simulink model "ARIES"  (R2024b)
settings: Solver=ode4  StartTime=0.0  StopTime=8*18601.8746  FixedStep=1e-1  RelTol=1e-3
model workspace (MAT data in the model file):
  BVH_bboxMax = Simulink.Parameter
  BVH_bboxMax.Value = [284.93805 4.355131 284.93805 278.0491 284.93805 284.65656 284.93805 139.47609 284.93805 284.93805 268.4671 268.4671 ... (24573 elements, 8191x3)]
  BVH_bboxMax.Complexity = 'real'
  BVH_bboxMax.Dimensions = [8191 3]
  BVH_bboxMax.DataType = 'auto'
  BVH_bboxMin = Simulink.Parameter
  BVH_bboxMin.Value = [-277.88974 -277.88974 -8.175628 -8.175628 -7.5725703 -7.2454505 -7.5725703 -7.5725703 128.49397 129.55234 128.49397 128.49397 ... (24573 elements, 8191x3)]
  BVH_bboxMin.Complexity = 'real'
  BVH_bboxMin.Dimensions = [8191 3]
  BVH_bboxMin.DataType = 'auto'
  BVH_fCount = Simulink.Parameter
  BVH_fCount.Value = [0 0 0 0 0 0 0 0 0 0 0 0 ... (8191 elements, 8191x1)]
  BVH_fCount.Complexity = 'real'
  BVH_fCount.Dimensions = [8191 1]
  BVH_fCount.DataType = 'int32'
  BVH_fStart = Simulink.Parameter
  BVH_fStart.Value = [0 0 0 0 0 0 0 0 0 0 0 0 ... (8191 elements, 8191x1)]
  BVH_fStart.Complexity = 'real'
  BVH_fStart.Dimensions = [8191 1]
  BVH_fStart.DataType = 'int32'
  BVH_faces = Simulink.Parameter
  BVH_faces.Value = [6744 6709 6709 6698 6730 6729 6745 6681 6682 6684 6684 6682 ... (74994 elements, 24998x3)]
  BVH_faces.Complexity = 'real'
  BVH_faces.Dimensions = [24998 3]
  BVH_faces.DataType = 'int32'
  BVH_left = Simulink.Parameter
  BVH_left.Value = [2 4098 4 2052 6 1030 8 520 10 266 12 140 ... (8191 elements, 8191x1)]
  BVH_left.Complexity = 'real'
  BVH_left.Dimensions = [8191 1]
  BVH_left.DataType = 'int32'
  BVH_normals = Simulink.Parameter
  BVH_normals.Value = [1 1 1 1 1 1 0 1 1 1 1 1 ... (74994 elements, 24998x3)]
  BVH_normals.Complexity = 'real'
  BVH_normals.Dimensions = [24998 3]
  BVH_normals.DataType = 'auto'
  BVH_right = Simulink.Parameter
  BVH_right.Value = [3 4099 5 2053 7 1031 9 521 11 267 13 141 ... (8191 elements, 8191x1)]
  BVH_right.Complexity = 'real'
  BVH_right.Dimensions = [8191 1]
  BVH_right.DataType = 'int32'
  BVH_vertexList = Simulink.Parameter
  BVH_vertexList.Value = [-118.90262 -122.20188 -116.06995 -125.190315 -127.74983 -122.412506 -131.21611 -134.88121 -129.40932 -138.59775 -133.93816 -136.61743 ... (37503 elements, 12501x3)]
  BVH_vertexList.Complexity = 'real'
  BVH_vertexList.Dimensions = [12501 3]
  BVH_vertexList.DataType = 'auto'
  WP_NWaypoints = Simulink.Parameter
  WP_NWaypoints.Value = 10
  WP_NWaypoints.Complexity = 'real'
  WP_NWaypoints.Dimensions = [1 1]
  WP_NWaypoints.DataType = 'int32'
  WP_STMArcs = Simulink.Parameter
  WP_STMArcs.Value = [1.1914426379 0.0471398153698 -0.00495904259985 0.00019235663522 7.56207628118e-05 -5.3765937279e-06 0.186775507685 0.598171523278 -0.000645694060378 0.000283020085834 -0.000320209392234 -4.9857312566e-07 ... (360 elements, 6x6x10)]
  WP_STMArcs.Complexity = 'real'
  WP_STMArcs.Dimensions = [6 6 10]
  WP_STMArcs.DataType = 'auto'
  WP_burnStrategy = Simulink.Parameter
  WP_burnStrategy.Value : enumeration (value not decoded)
  WP_burnStrategy.Complexity = 'real'
  WP_burnStrategy.Dimensions = [1 1]
  WP_burnStrategy.DataType = 'Enum: burnStrategyVariant'
  WP_dtArc = Simulink.Parameter
  WP_dtArc.Value = 1860.18745936
  WP_dtArc.Complexity = 'real'
  WP_dtArc.Dimensions = [1 1]
  WP_dtArc.DataType = 'auto'
  WP_proxRadius = Simulink.Parameter
  WP_proxRadius.Value = 200
  WP_proxRadius.Complexity = 'real'
  WP_proxRadius.Dimensions = [1 1]
  WP_proxRadius.DataType = 'auto'
  WP_waypointPosition = Simulink.Parameter
  WP_waypointPosition.Value = [350  0  0; 283.155948031  205.724838302  0; 108.155948031  332.869780703  0; -108.155948031  332.869780703  0; -283.155948031  205.724838302  0; -350  4.28626379702e-14  0; -283.155948031  -205.724838302  0; -108.155948031  -332.869780703  0; 108.155948031  -332.869780703  0; 283.155948031  -205.724838302  0]
  WP_waypointPosition.Complexity = 'real'
  WP_waypointPosition.Dimensions = [10 3]
  WP_waypointPosition.DataType = 'auto'
  WP_waypointVelocity = Simulink.Parameter
  WP_waypointVelocity.Value = [0  -0.0241739331755  0; 0.0142090814104  -0.0195571227598  0; 0.022990776671  -0.0074701561721  0; 0.022990776671  0.0074701561721  0; 0.0142090814104  0.0195571227598  0; 2.96045298861e-18  0.0241739331755  0; -0.0142090814104  0.0195571227598  0; -0.022990776671  0.0074701561721  0; -0.022990776671  -0.0074701561721  0; -0.0142090814104  -0.0195571227598  0]
  WP_waypointVelocity.Complexity = 'real'
  WP_waypointVelocity.Dimensions = [10 3]
  WP_waypointVelocity.DataType = 'auto'
  asteroidAngularVelocity = Simulink.Parameter
  asteroidAngularVelocity.Value = [0; 0; 0.00040684]
  asteroidAngularVelocity.Complexity = 'real'
  asteroidAngularVelocity.Dimensions = [3 1]
  asteroidAngularVelocity.DataType = 'auto'
values from neighbouring files (symbols this model uses):
  actuators = actuatorsConfig()    [mainMontecarlo.m]    (also in mainSimulator.m)
  environment = environmentConfig(gravDataPath)    [mainMontecarlo.m]    (also in mainSimulator.m; mainWaypointGenerator.m = environmentConfig(gravDataPath, true))
  gravAtt = Simulink.Parameter(environment.gravStruct.gravAtt)    [mainSimulator.m]    (also in mainWaypointGenerator.m)
  init = initConditionConfig(control)    [mainMontecarlo.m]    (also in mainSimulator.m)
  simulation = simulationConfig()    [mainMontecarlo.m]    (also in mainSimulator.m = simulationConfig(control, environment))
undefined symbols (not defined in the file or in its folder): control, magnitude, spacecraft
libraries: matrix_library x14, aerolibutil x4, sharedutil x2, sharedtransform x2, simulink x2
(part 1 of 2)
settings Model: SimulationMode=rapid-accelerator  PauseTimes=10  ExtModeTrigDuration=100  Creator=pierb  LastModifiedBy=pierb
settings SolverCC: MinimalZcImpactIntegration=on
settings OptimizationCC: UseDivisionForNetSlopeComputation=on  GainParamInheritBuiltInType=on  UseFloatMulNetSlope=on  UseSpecifiedMinMax=on  PassReuseOutputArgsAs=Individual arguments  ZeroExternalMemoryAtStartup=off  ZeroInternalMemoryAtStartup=off  NoFixptDivByZeroProtection=on  EfficientFloat2IntCast=on  LifeSpan=1  MaxStackSize=10000000  OptimizeBlockOrder=speed  DifferentSizesBufferReuse=on  EfficientTunableParamExpr=on
settings DebuggingCC: ReadBeforeWriteMsg=DisableAll  WriteAfterWriteMsg=DisableAll  WriteAfterReadMsg=DisableAll  MultiTaskDSMMsg=none  ParameterTunabilityLossMsg=error
settings HardwareCC: ProdBitPerInt=16  ProdBitPerPointer=16  ProdBitPerSizeT=16  ProdBitPerPtrDiffT=16  ProdLargestAtomicFloat=None  ProdWordSize=16  ProdLongLongMode=on  ProdHWDeviceType=STMicroelectronics->ST10/Super10
settings ModelReferenceCC: UpdateModelReferenceTargets=IfOutOfDate
settings SFSimCC: SFSimEcho=off  MATLABDynamicMemAlloc=off
settings RTWCC: Description=Embedded Coder  SystemTargetFile=ert.tlc  GenCodeOnly=on  PackageGeneratedCodeAndArtifacts=on  TemplateMakefile=ert_default_tmf  GenerateReport=on  Toolchain=CMake  BuildConfiguration=Faster Runs  LaunchReport=on  CodeProfilingSaveOptions=AllData  DataTypeReplacement=CDataTypesFixedWidth  TargetLang=C++  CheckMdlBeforeBuild=Warning
settings CodeAppCC: ForceParamTrailComments=on  IgnoreCustomStorageClasses=off  OperatorAnnotations=on  SimulinkDataObjDesc=on  SFDataObjDesc=on  CustomSymbolStrGlobalVar=rt$N$M  CustomSymbolStrType=$N$M  CustomSymbolStrFcn=$N$M$F  CustomSymbolStrMacro=$N$M  InsertBlockDesc=on
settings ERTTargetCC: TargetLangStandard=C++11 (ISO)  GenerateSampleERTMain=on  IncludeMdlTerminateFcn=off  CombineSignalStateStructs=on  SuppressErrorStatus=on  CodeInterfacePackaging=C++ class  SupportNonFinite=off  SupportComplex=off  InlinedParameterPlacement=Hierarchical  RootIOFormat=Structure reference  ERTCustomFileTemplate=example_file_process.tlc  ERTFilePackagingFormat=CompactWithDataFile  MaxIdInt64=INT64_MAX  MinIdInt64=INT64_MIN  MaxIdUint64=UINT64_MAX  MaxIdInt32=INT32_MAX  MinIdInt32=INT32_MIN  MaxIdUint32=UINT32_MAX  MaxIdInt16=INT16_MAX  MinIdInt16=INT16_MIN  MaxIdUint16=UINT16_MAX  MaxIdInt8=INT8_MAX  MinIdInt8=INT8_MIN  MaxIdUint8=UINT8_MAX

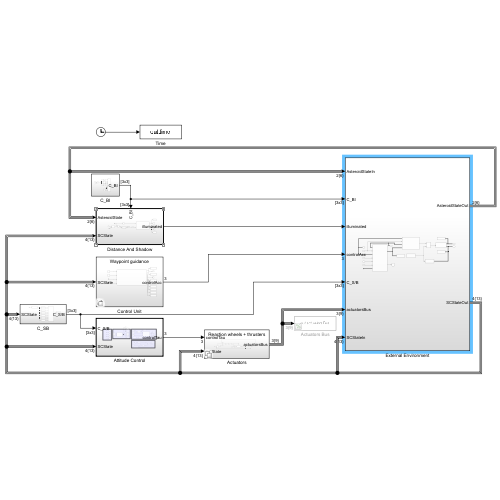
[thumbnail: Simulink's stored preview of the top-level diagram]
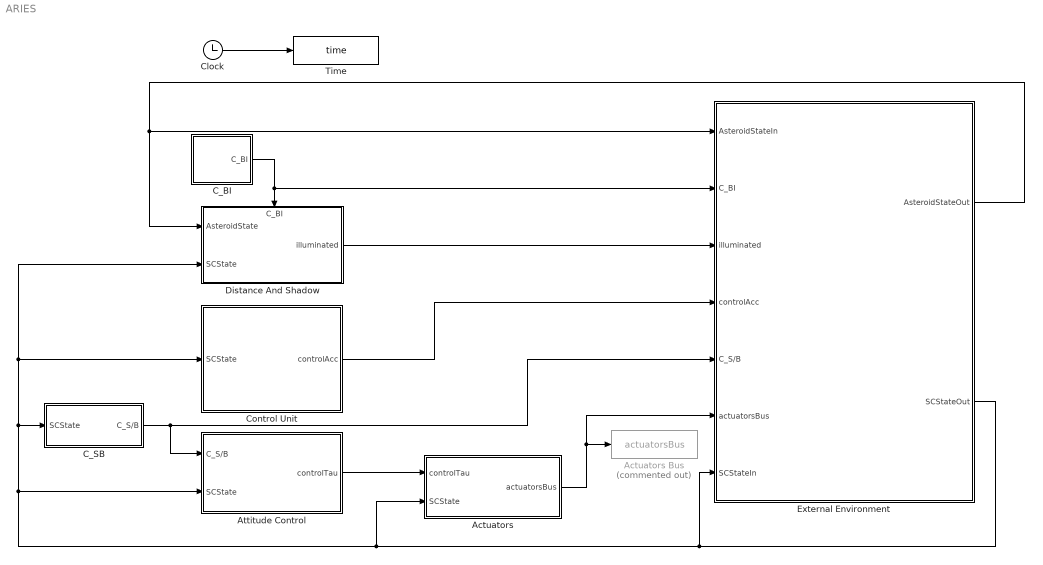
== system ARIES ==
  Actuators : Subsystem  Variant=on  VariantControl=Actuators
  Actuators Bus : ToWorkspace  Commented=on  VariableName=actuatorsBus  SaveFormat=Timeseries  SampleTime=-1
  Attitude Control : Subsystem  TreatAsAtomicUnit=on  SystemSampleTime=1
  C_BI : Subsystem
  C_SB : Subsystem
  Clock : Clock
  Control Unit : Subsystem  Variant=on  VariantControl=Orbit Keeping Control  AllowFlexibleInterface=off
  Distance And Shadow : Subsystem  TreatAsAtomicUnit=on  SystemSampleTime=1
      settings: PortSchema="{\"entries\":[{\"content\":{\"sides\":[{\"content\":{\"connectorIds\":[\"In1\",\"In2\"]},\"type\":\"ConnectorPlacement.EquallySpacedRectSide\",\"uuid\":\"8e6886da-42bf-46c1-bf35-0160fb199749\"},{\"content\":{\"connectorIds\":[\"Out1\"],\"side\":\"RIGHT\"},\"type\":\"ConnectorPlacement.EquallySpacedRectSide\",\"uuid\":\"a834982d-232b-47fa-a58c-d8537adbd461\"},{\"content\":{\"connectorIds\":[\"In3\"],\"side\":\"TOP\"},\"type\":\"ConnectorPlacement.EquallySpacedRectSide\",\"uuid\":\"dc81c1cd-5046-42e0-b637-5e4c02a19139\"}]},\"type\":\"ConnectorPlacement.EquallySpacedConnector\",\"uuid\":\"7ef6c02e-89ea-4520-8812-5e1f6d5bbb11\"}],\"packageUris\":[\"http://schema.mathworks.com/mf0/Connector/R2020b\"],\"version\":\"1.0\"}"
  External Environment : Subsystem
  Time : ToWorkspace  VariableName=time  SampleTime=-1
  wires:
  Clock/1 -> Time/1
  C_BI/1(C_BI) -> Distance And Shadow/3(C_BI), External Environment/2(C_BI)
  External Environment/1(AsteroidStateOut) -> External Environment/1(AsteroidStateIn), Distance And Shadow/1(AsteroidState)
  External Environment/2(SCStateOut) -> Actuators/2(SCState), Distance And Shadow/2(SCState), Control Unit/1(SCState), C_SB/1(SCState), Attitude Control/2(SCState), External Environment/7(SCStateIn)
  C_SB/1(C_S/B) -> Attitude Control/1(C_S/B), External Environment/5(C_S/B)
  Attitude Control/1(controlTau) -> Actuators/1(controlTau)
  Actuators/1(actuatorsBus) -> External Environment/6(actuatorsBus), Actuators Bus/1
  Distance And Shadow/1(illuminated) -> External Environment/3(illuminated)
  Control Unit/1(controlAcc) -> External Environment/4(controlAcc)

== system ARIES/Actuators ==
  controlTau : Inport
  SCState : Inport  Port=2
  NO actuators : Subsystem  VariantControl="simulation.variants.attActuator == \"NO_ACTUATOR\""
  Reaction wheels + thrusters : Subsystem  VariantControl="simulation.variants.attActuator == \"REACTION_WHEELS_PYRAMID\""
  actuatorsBus : Outport

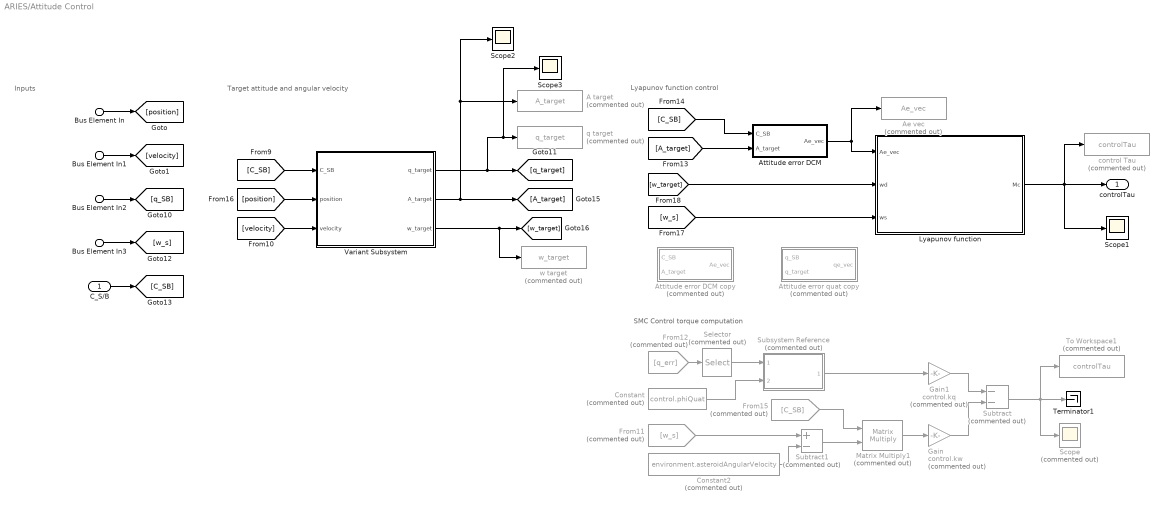
== system ARIES/Attitude Control ==
  note: Target attitude and angular velocity
  note: Lyapunov function control
  note: SMC Control torque computation
  note: Inputs
  C_S/B : Inport
  Bus Element In : Inport  Port=2  PortName=SCState  Element=position
  Bus Element In1 : Inport  Port=2  PortName=SCState  Element=velocity
  Bus Element In2 : Inport  Port=2  PortName=SCState  Element=q_SB
  Bus Element In3 : Inport  Port=2  PortName=SCState  Element=ang_velocity
  A target : ToWorkspace  Commented=on  VariableName=A_target  SaveFormat=Timeseries  SampleTime=-1
  Ae vec : ToWorkspace  Commented=on  VariableName=Ae_vec  SaveFormat=Timeseries  SampleTime=-1
  Attitude error DCM : Subsystem
  Attitude error DCM copy : Subsystem  Commented=on
  Attitude error quat copy : Subsystem  Commented=on
  Constant : Constant  Commented=on  Value=control.phiQuat
  Constant2 : Constant  Commented=on  Value=environment.asteroidAngularVelocity
  From11 : From  Commented=on  GotoTag=w_s
  From12 : From  Commented=on  GotoTag=q_err
  From15 : From  Commented=on  GotoTag=C_SB
  Gain : Gain  Commented=on  Gain=control.kw
  Gain1 : Gain  Commented=on  Gain=control.kq
  Lyapunov function : Subsystem
  Matrix Multiply1 : Product  Commented=on  Multiplication=Matrix(*)
  Scope : Scope  Commented=on
  Scope1 : Scope
  Scope2 : Scope
  Scope3 : Scope
  Selector : Selector  Commented=on  InputPortWidth=4  IndexOptions=Index vector (dialog)  Indices=[2:4]  OutputSizes=1
  Subsystem Reference : Subsystem  Commented=on  ReferencedSubsystem=saturation
  Subtract : Sum  Commented=on  Inputs=--
  Subtract1 : Sum  Commented=on  Inputs=+-
  Terminator1 : Terminator
  To Workspace1 : ToWorkspace  Commented=on  VariableName=controlTau  SaveFormat=Timeseries  SampleTime=-1
  Variant Subsystem : Subsystem  Variant=on
  control Tau : ToWorkspace  Commented=on  VariableName=controlTau  SaveFormat=Timeseries  SampleTime=-1
  q target : ToWorkspace  Commented=on  VariableName=q_target  SaveFormat=Timeseries  SampleTime=-1
  w target : ToWorkspace  Commented=on  VariableName=w_target  SaveFormat=Timeseries  SampleTime=-1
  controlTau : Outport
  wires:
  Bus Element In1/1 -> [velocity]
  Bus Element In/1 -> [position]
  Bus Element In2/1 -> [q_SB]
  Bus Element In3/1 -> [w_s]
  From11/1 -> Subtract1/1
  Gain/1 -> Subtract/2
  Subsystem Reference/1 -> Gain1/1
  From12/1 -> Selector/1
  Selector/1 -> Subsystem Reference/1
  Constant/1 -> Subsystem Reference/2
  Gain1/1 -> Subtract/1
  Subtract1/1 -> Matrix Multiply1/2
  Constant2/1 -> Subtract1/2
  Subtract/1 -> To Workspace1/1, Terminator1/1, Scope/1
  From15/1 -> Matrix Multiply1/1
  Matrix Multiply1/1 -> Gain/1
  [C_SB] -> Attitude error DCM/1(C_SB)
  C_S/B/1 -> [C_SB]
  [A_target] -> Attitude error DCM/2(A_target)
  Attitude error DCM/1(Ae_vec) -> Ae vec/1, Lyapunov function/1(Ae_vec)
  Lyapunov function/1(Mc) -> control Tau/1, controlTau/1, Scope1/1
  [w_s] -> Lyapunov function/3(ws)
  [w_target] -> Lyapunov function/2(wd)
  [C_SB] -> Variant Subsystem/1(C_SB)
  [position] -> Variant Subsystem/2(position)
  [velocity] -> Variant Subsystem/3(velocity)
  Variant Subsystem/1(q_target) -> Scope3/1, q target/1, [q_target]
  Variant Subsystem/2(A_target) -> [A_target], Scope2/1, A target/1
  Variant Subsystem/3(w_target) -> w target/1, [w_target]

== system ARIES/C_BI ==
  CBIMat : ToWorkspace  VariableName=C_BI  SaveFormat=Timeseries  SampleTime=-1
  Clock : Clock
  Constant : Constant
  Constant1 : Constant  Value=0
  Constant2 : Constant  Value=0
  Cos : Trigonometry  Operator=cos
  Cos1 : Trigonometry  Operator=cos
  Cos2 : Trigonometry
  Cos3 : Trigonometry
  Gain2 : Gain  Gain=-1
  Product : Product
  Subsystem Reference : Subsystem  ReferencedSubsystem=Create3x3Matrix
  wb : Constant  Value=environment.asteroidAngularVelocity(end)
  C_BI : Outport
  wires:
  wb/1 -> Product/1
  Constant2/1 -> Subsystem Reference/3
  Clock/1 -> Product/2
  Constant/1 -> Subsystem Reference/9
  Constant1/1 -> Subsystem Reference/7, Subsystem Reference/6, Subsystem Reference/8
  Cos/1 -> Subsystem Reference/1
  Cos1/1 -> Subsystem Reference/5
  Subsystem Reference/1 -> CBIMat/1, C_BI/1
  Product/1 -> Cos1/1, Cos3/1, Cos2/1, Cos/1
  Cos2/1 -> Subsystem Reference/2
  Cos3/1 -> Gain2/1
  Gain2/1 -> Subsystem Reference/4

== system ARIES/C_SB ==
  Bus Element In : Inport  PortName=SCState  Element=q_SB
  A11 : Subsystem
  A12 : Subsystem
  A13 : Subsystem
  A21 : Subsystem
  A22 : Subsystem
  A23 : Subsystem
  A31 : Subsystem
  A32 : Subsystem
  A33 : Subsystem
  CSBMat : ToWorkspace  VariableName=C_SB  SaveFormat=Timeseries  SampleTime=-1
  Create3x3Matrix : Subsystem  ReferencedSubsystem=Create3x3Matrix
  quatNormalize : Subsystem  ReferencedSubsystem=quatNormalize
  C_S/B : Outport  Unit=1  PortDimensions=[3,3]  InitialOutput=0  VectorParamsAs1DForOutWhenUnconnected=off
  wires:
  Bus Element In/1 -> quatNormalize/1
  A13/1(A13) -> Create3x3Matrix/3
  A33/1(A33) -> Create3x3Matrix/9
  A22/1(A22) -> Create3x3Matrix/5
  A23/1(A23) -> Create3x3Matrix/6
  A11/1(A11) -> Create3x3Matrix/1
  A21/1(A21) -> Create3x3Matrix/4
  A31/1(A31) -> Create3x3Matrix/7
  quatNormalize/1 -> A11/1(qNormalized), A12/1(qNormalized), A13/1(qNormalized), A21/1(qNormalized), A22/1(qNormalized), A23/1(qNormalized), A31/1(qNormalized), A32/1(qNormalized), A33/1(qNormalized)
  A12/1(A12) -> Create3x3Matrix/2
  Create3x3Matrix/1 -> CSBMat/1, C_S/B/1
  A32/1(A32) -> Create3x3Matrix/8

== system ARIES/Control Unit ==
  SCState : Inport
  No Control : Subsystem  TreatAsAtomicUnit=on  SystemSampleTime=1  VariantControl=ctrlVar == controlVariant.NO_CONTROL
  Orbit Keeping Control : Subsystem  TreatAsAtomicUnit=on  SystemSampleTime=1  VariantControl=ctrlVar == controlVariant.ORBIT_KEEPING
  Waypoint guidance : Subsystem  SystemSampleTime=str2num(simulation.simulationTimeStep)  VariantControl=ctrlVar== controlVariant.WAYPOINT
  controlAcc : Outport

== system ARIES/Distance And Shadow ==
  Bus Element In3 : Inport  PortName=AsteroidState  Element=position
  Bus Element In : Inport  Port=2  PortName=SCState  Element=position
  C_BI : Inport  Port=3
  Add : Sum
  Distance : ToWorkspace  VariableName=distance  SaveFormat=Timeseries  SampleTime=-1
  Divide : Product  Inputs=*/
  Illuminated State : ToWorkspace  VariableName=illuminated  SaveFormat=Timeseries  SampleTime=-1
  Matrix Multiply : Product  Multiplication=Matrix(*)
  Reshape : Reshape  OutputDimensionality=Row vector (2-D)
  Reshape1 : Reshape  OutputDimensionality=Row vector (2-D)
  Scope : Scope
  Scope1 : Scope
  Subsystem Reference : Subsystem  ReferencedSubsystem=VectorNorm
  pointToMeshDistanceAndShadow : MATLAB Function  TreatAsAtomicUnit=on
  illuminated : Outport
  wires:
  C_BI/1 -> Matrix Multiply/1
  Reshape/1 -> pointToMeshDistanceAndShadow/1(position)
  Add/1 -> Divide/1, Subsystem Reference/1
  Bus Element In/1 -> Reshape/1, Add/1
  Bus Element In3/1 -> Matrix Multiply/2
  Matrix Multiply/1 -> Add/2
  Subsystem Reference/1 -> Divide/2
  Divide/1 -> Reshape1/1
  Reshape1/1 -> pointToMeshDistanceAndShadow/2(sunDir)
  pointToMeshDistanceAndShadow/1(dist) -> Distance/1, Scope/1
  pointToMeshDistanceAndShadow/2(illuminated) -> illuminated/1, Illuminated State/1, Scope1/1

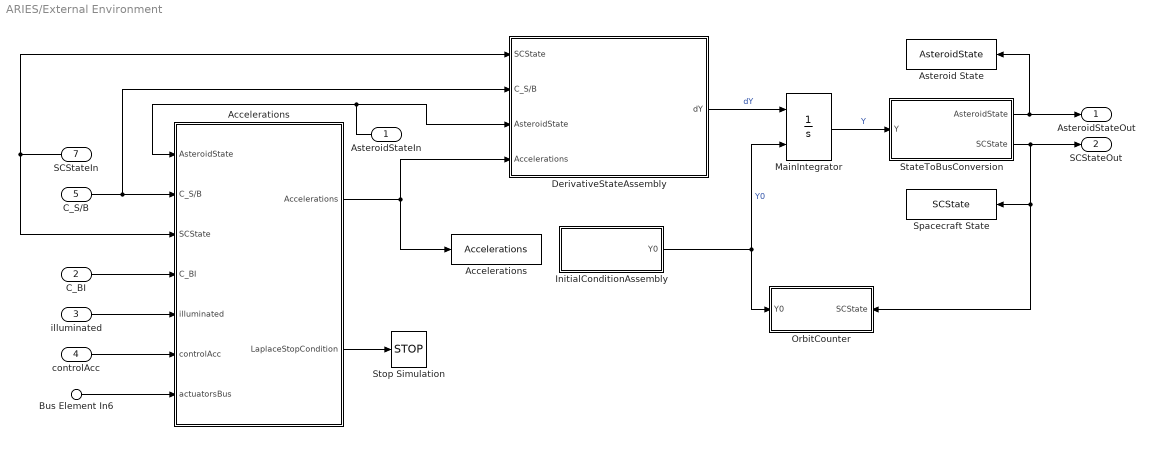
== system ARIES/External Environment ==
  AsteroidStateIn : Inport
  C_BI : Inport  Port=2
  illuminated : Inport  Port=3
  controlAcc : Inport  Port=4
  C_S/B : Inport  Port=5
  Bus Element In6 : Inport  Port=6  PortName=actuatorsBus
  SCStateIn : Inport  Port=7
  Accelerations : Subsystem
  "Accelerations " : ToWorkspace  VariableName=Accelerations  SaveFormat=Timeseries  SampleTime=-1
  Asteroid State : ToWorkspace  VariableName=AsteroidState  SaveFormat=Timeseries  SampleTime=-1
  DerivativeStateAssembly : Subsystem
  InitialConditionAssembly : Subsystem
  MainIntegrator : Integrator  InitialConditionSource=external
  OrbitCounter : Subsystem
      settings: PortSchema="{\"entries\":[{\"content\":{\"sides\":[{\"content\":{\"connectorIds\":[\"In1\"]},\"type\":\"ConnectorPlacement.EquallySpacedRectSide\",\"uuid\":\"c18985fd-cd07-4158-af1a-24c086147cad\"},{\"content\":{\"connectorIds\":[\"In2\"],\"side\":\"RIGHT\"},\"type\":\"ConnectorPlacement.EquallySpacedRectSide\",\"uuid\":\"b4d0cf3d-3086-43c8-9feb-6aa9351d55e5\"},{\"content\":{\"side\":\"TOP\"},\"type\":\"ConnectorPlacement.EquallySpacedRectSide\",\"uuid\":\"2e268a01-377c-4312-8f82-9d41e9830e6b\"}]},\"type\":\"ConnectorPlacement.EquallySpacedConnector\",\"uuid\":\"37a36cff-a92f-4c53-8284-dfeb1ddda685\"}],\"packageUris\":[\"http://schema.mathworks.com/mf0/Connector/R2020b\"],\"version\":\"1.0\"}"
  Spacecraft State : ToWorkspace  VariableName=SCState  SaveFormat=Timeseries  SampleTime=-1
  StateToBusConversion : Subsystem
  Stop Simulation : Stop
  AsteroidStateOut : Outport
  SCStateOut : Outport  Port=2
  wires:
  Accelerations/2(LaplaceStopCondition) -> Stop Simulation/1
  AsteroidStateIn/1 -> Accelerations/1(AsteroidState), DerivativeStateAssembly/3(AsteroidState)
  Accelerations/1(Accelerations) -> "Accelerations "/1, DerivativeStateAssembly/4(Accelerations)
  StateToBusConversion/2(SCState) -> OrbitCounter/2(SCState), Spacecraft State/1, SCStateOut/1
  C_S/B/1 -> DerivativeStateAssembly/2(C_S/B), Accelerations/2(C_S/B)
  MainIntegrator/1 -> StateToBusConversion/1(Y)  "Y"
  InitialConditionAssembly/1(Y0) -> MainIntegrator/2, OrbitCounter/1(Y0)  "Y0"
  DerivativeStateAssembly/1(dY) -> MainIntegrator/1  "dY"
  C_BI/1 -> Accelerations/4(C_BI)
  illuminated/1 -> Accelerations/5(illuminated)
  SCStateIn/1 -> DerivativeStateAssembly/1(SCState), Accelerations/3(SCState)
  controlAcc/1 -> Accelerations/6(controlAcc)
  Bus Element In6/1 -> Accelerations/7(actuatorsBus)
  StateToBusConversion/1(AsteroidState) -> Asteroid State/1, AsteroidStateOut/1

== system ARIES/Actuators/NO actuators ==
  controlTau : Inport
  Gain : Gain  Gain=-1
  Reshape : Reshape
  Reshape1 : Reshape
  Zero : Constant  Value=zeros(3,1)  OutDataTypeStr=Inherit: Inherit via back propagation
  Zero1 : Constant  Value=zeros(3,1)  OutDataTypeStr=Inherit: Inherit via back propagation
  Bus Element Out1 : Outport  PortName=actuatorsBus  Element=rw.dhr
  Bus Element Out2 : Outport  PortName=actuatorsBus  Element=rw.hr
  Bus Element Out3 : Outport  PortName=actuatorsBus  Element=attThruster.tauDesat
  wires:
  controlTau/1 -> Gain/1
  Zero1/1 -> Reshape/1
  Zero/1 -> Reshape1/1
  Reshape/1 -> Bus Element Out3/1
  Reshape1/1 -> Bus Element Out2/1
  Gain/1 -> Bus Element Out1/1

== system ARIES/Actuators/Reaction wheels + thrusters ==
  controlTau : Inport
  Bus Element In2 : Inport  Port=2  PortName=SCState  Element=ang_velocity
  Add : Sum  Inputs=+++
  Constant : Constant  Value=init.hr0
  Cross Product : matrix_library/Cross Product
  Gain : Gain  Gain=-1
  Integrator : Integrator  InitialConditionSource=external
  Memory : Memory
  Reshape : Reshape
  Reshape1 : Reshape
  Reshape2 : Reshape
  dhr_sat : Saturate  UpperLimit=actuators.rw.hrDotMax_total * ones(3,1)  LowerLimit=-actuators.rw.hrDotMax_total * ones(3,1)
  hr_sat : Subsystem
  tauDesatComputation : Subsystem
  Bus Element Out1 : Outport  PortName=actuatorsBus  Element=rw.dhr
  Bus Element Out2 : Outport  PortName=actuatorsBus  Element=rw.hr
  Bus Element Out3 : Outport  PortName=actuatorsBus  Element=attThruster.tauDesat
  wires:
  Reshape1/1 -> tauDesatComputation/1(hr), Bus Element Out2/1, Cross Product/2
  Gain/1 -> dhr_sat/1
  Add/1 -> Gain/1
  controlTau/1 -> Add/2
  Bus Element In2/1 -> Cross Product/1
  Cross Product/1 -> Add/3
  Integrator/1 -> hr_sat/1(hr)
  Constant/1 -> Integrator/2
  dhr_sat/1 -> Reshape2/1
  Reshape2/1 -> Bus Element Out1/1, Integrator/1
  hr_sat/1(hr_sat) -> Reshape1/1
  tauDesatComputation/1(tauDesat) -> Reshape/1
  Reshape/1 -> Add/1, Bus Element Out3/1
  tauDesatComputation/2(active) -> Memory/1
  Memory/1 -> tauDesatComputation/2(activePrev)

== system ARIES/Attitude Control/Attitude error DCM ==
  C_SB : Inport
  A_target : Inport  Port=2
  MATLAB Function : MATLAB Function  TreatAsAtomicUnit=on
  Matrix Multiply : Product  Multiplication=Matrix(*)
  Transpose : Math  Operator=transpose
  Ae_vec : Outport
  wires:
  A_target/1 -> Transpose/1
  C_SB/1 -> Matrix Multiply/1
  Transpose/1 -> Matrix Multiply/2
  MATLAB Function/1(Ae_vec) -> Ae_vec/1
  Matrix Multiply/1 -> MATLAB Function/1(Ce)  "Ae"

== system ARIES/Attitude Control/Attitude error DCM copy ==
  C_SB : Inport
  A_target : Inport  Port=2
  MATLAB Function : MATLAB Function  TreatAsAtomicUnit=on
  Matrix Multiply : Product  Multiplication=Matrix(*)
  Transpose : Math  Operator=transpose
  Ae_vec : Outport
  wires:
  Matrix Multiply/1 -> MATLAB Function/1(Ce)  "Ae"
  MATLAB Function/1(Ae_vec) -> Ae_vec/1
  Transpose/1 -> Matrix Multiply/2
  C_SB/1 -> Matrix Multiply/1
  A_target/1 -> Transpose/1

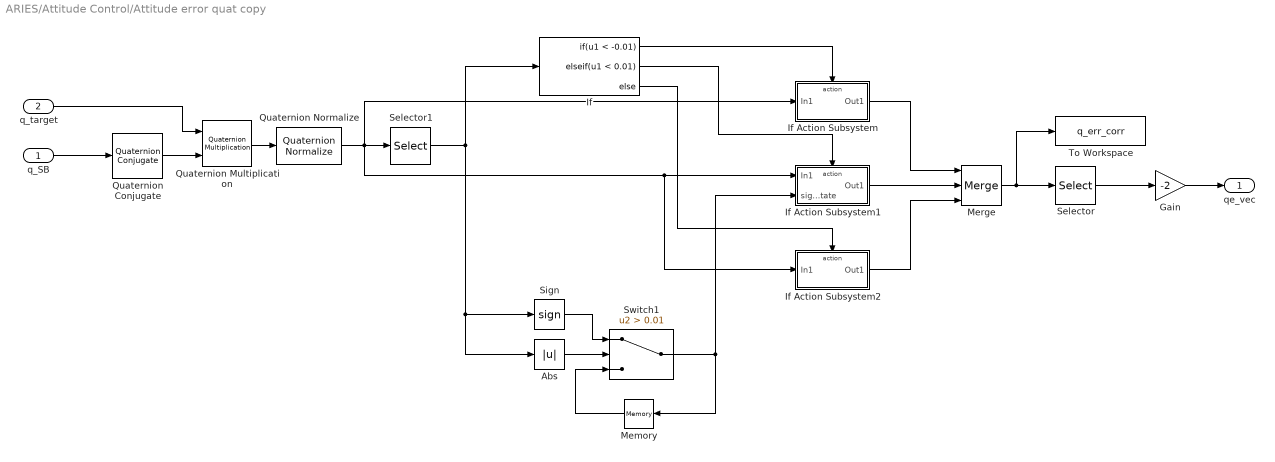
== system ARIES/Attitude Control/Attitude error quat copy ==
  q_SB : Inport
  q_target : Inport  Port=2
  Abs : Abs  SaturateOnIntegerOverflow=off
  Gain : Gain  Gain=-2
  If : If  IfExpression=u1 < -0.01  ElseIfExpressions=u1 < 0.01
  If Action Subsystem : Subsystem  TreatAsAtomicUnit=on
  If Action Subsystem1 : Subsystem  TreatAsAtomicUnit=on
  If Action Subsystem2 : Subsystem  TreatAsAtomicUnit=on
  Memory : Memory  InitialCondition=1
  Merge : Merge  Inputs=3
  Quaternion Conjugate : aerolibutil/Quaternion Conjugate
  Quaternion Multiplication : aerolibutil/Quaternion Multiplication
  Quaternion Normalize : sharedutil/Quaternion Normalize  aMode=aMode
  Selector : Selector  InputPortWidth=4  IndexOptions=Index vector (dialog)  Indices=[2:4]  OutputSizes=1
  Selector1 : Selector  InputPortWidth=4  IndexOptions=Index vector (dialog)  Indices=1  OutputSizes=1
  Sign : Signum
  Switch1 : Switch  Criteria=u2 > Threshold  Threshold=0.01  SaturateOnIntegerOverflow=off  InputSameDT=off
  To Workspace : ToWorkspace  VariableName=q_err_corr  SaveFormat=Timeseries  SampleTime=-1
  qe_vec : Outport
  wires:
  Selector/1 -> Gain/1
  Gain/1 -> qe_vec/1
  Quaternion Normalize/1 -> If Action Subsystem2/1(In1), If Action Subsystem1/1(In1), If Action Subsystem/1(In1), Selector1/1
  Merge/1 -> To Workspace/1, Selector/1
  Quaternion Multiplication/1 -> Quaternion Normalize/1
  Quaternion Conjugate/1 -> Quaternion Multiplication/2
  q_SB/1 -> Quaternion Conjugate/1
  q_target/1 -> Quaternion Multiplication/1
  Abs/1 -> Switch1/2
  Sign/1 -> Switch1/1
  Switch1/1 -> If Action Subsystem1/2(sign_state), Memory/1
  Memory/1 -> Switch1/3
  Selector1/1 -> Sign/1, Abs/1, If/1
  If/1 -> If Action Subsystem/Action
  If/2 -> If Action Subsystem1/Action
  If/3 -> If Action Subsystem2/Action
  If Action Subsystem/1(Out1) -> Merge/1
  If Action Subsystem1/1(Out1) -> Merge/2
  If Action Subsystem2/1(Out1) -> Merge/3

== system ARIES/Attitude Control/Lyapunov function ==
  Ae_vec : Inport
  wd : Inport  Port=2
  ws : Inport  Port=3
  Add : Sum  Inputs=+++
  Cross Product : matrix_library/Cross Product
  I_mat : Gain  Gain=spacecraft.I_mat  Multiplication=Matrix(K*u)
  Reshape : Reshape
  Subtract : Sum  Inputs=+-
  katt : Gain  Gain=control.katt
  kw : Gain  Gain=control.kw
  Mc : Outport
  wires:
  wd/1 -> Subtract/1
  ws/1 -> Subtract/2, Cross Product/1, I_mat/1
  Subtract/1 -> kw/1
  Ae_vec/1 -> katt/1
  I_mat/1 -> Cross Product/2
  katt/1 -> Add/1
  kw/1 -> Add/2
  Cross Product/1 -> Add/3
  Add/1 -> Reshape/1
  Reshape/1 -> Mc/1

== system ARIES/Attitude Control/Variant Subsystem ==
  C_SB : Inport
  position : Inport  Port=2
  velocity : Inport  Port=3
  INERTIAL : Subsystem  VariantControl="simulation.variants.attTarget == \"INERTIAL\""
  ZENITH : Subsystem  VariantControl="simulation.variants.attTarget == \"ZENITH_POINTING\""
  q_target : Outport
  A_target : Outport  Port=2
  w_target : Outport  Port=3

== system ARIES/C_SB/A11 ==
  qNormalized : Inport
  Demux : Demux
  Product{,1..3} (4 alike) : Product  RndMeth=Zero
  Sum : Sum  Inputs=++--
  A11 : Outport  VectorParamsAs1DForOutWhenUnconnected=off
  wires:
  Demux/3 -> Product1/1, Product1/2
  Demux/4 -> Product/1, Product/2
  Sum/1 -> A11/1
  Product/1 -> Sum/4
  Product1/1 -> Sum/3
  Demux/1 -> Product3/1, Product3/2
  qNormalized/1 -> Demux/1
  Product3/1 -> Sum/1
  Demux/2 -> Product2/1, Product2/2
  Product2/1 -> Sum/2

== system ARIES/C_SB/A12 ==
  qNormalized : Inport
  Demux : Demux
  Gain : Gain  Gain=2
  Product2 : Product  RndMeth=Zero
  Product3 : Product  RndMeth=Zero
  Sum : Sum  Inputs=|++
  A12 : Outport  VectorParamsAs1DForOutWhenUnconnected=off
  wires:
  Sum/1 -> Gain/1
  Gain/1 -> A12/1
  Demux/4 -> Product3/1
  qNormalized/1 -> Demux/1
  Product3/1 -> Sum/1
  Product2/1 -> Sum/2
  Demux/3 -> Product2/2
  Demux/2 -> Product2/1
  Demux/1 -> Product3/2

== system ARIES/C_SB/A13 ==
  qNormalized : Inport
  Demux : Demux
  Gain : Gain  Gain=2
  Product1 : Product  RndMeth=Zero
  Product2 : Product  RndMeth=Zero
  Sum : Sum  Inputs=|-+
  A13 : Outport  VectorParamsAs1DForOutWhenUnconnected=off
  wires:
  Demux/1 -> Product1/1
  Demux/4 -> Product2/2
  Product2/1 -> Sum/2
  Demux/3 -> Product1/2
  Sum/1 -> Gain/1
  Gain/1 -> A13/1
  Demux/2 -> Product2/1
  Product1/1 -> Sum/1
  qNormalized/1 -> Demux/1

== system ARIES/C_SB/A21 ==
  qNormalized : Inport
  Demux : Demux
  Gain : Gain  Gain=2
  Product2 : Product  RndMeth=Zero
  Product3 : Product  RndMeth=Zero
  Sum : Sum  Inputs=|-+
  A21 : Outport  VectorParamsAs1DForOutWhenUnconnected=off
  wires:
  Demux/3 -> Product2/2
  Demux/2 -> Product2/1
  Sum/1 -> Gain/1
  Gain/1 -> A21/1
  Demux/4 -> Product3/1
  Product2/1 -> Sum/2
  Demux/1 -> Product3/2
  Product3/1 -> Sum/1
  qNormalized/1 -> Demux/1

== system ARIES/C_SB/A22 ==
  qNormalized : Inport
  Demux : Demux
  Product{,1..3} (4 alike) : Product  RndMeth=Zero
  Sum : Sum  Inputs=+-+-
  A22 : Outport  VectorParamsAs1DForOutWhenUnconnected=off
  wires:
  Demux/3 -> Product1/1, Product1/2
  Demux/4 -> Product/1, Product/2
  Sum/1 -> A22/1
  Product/1 -> Sum/4
  Product1/1 -> Sum/3
  Demux/1 -> Product3/1, Product3/2
  qNormalized/1 -> Demux/1
  Product3/1 -> Sum/1
  Demux/2 -> Product2/1, Product2/2
  Product2/1 -> Sum/2

== system ARIES/C_SB/A23 ==
  qNormalized : Inport
  Demux : Demux
  Gain : Gain  Gain=2
  Product1 : Product  RndMeth=Zero
  Product2 : Product  RndMeth=Zero
  Sum : Sum  Inputs=|++
  A23 : Outport  VectorParamsAs1DForOutWhenUnconnected=off
  wires:
  Demux/2 -> Product1/2
  Product1/1 -> Sum/1
  Gain/1 -> A23/1
  qNormalized/1 -> Demux/1
  Product2/1 -> Sum/2
  Sum/1 -> Gain/1
  Demux/1 -> Product1/1
  Demux/3 -> Product2/1
  Demux/4 -> Product2/2

== system ARIES/C_SB/A31 ==
  qNormalized : Inport
  Demux : Demux
  Gain : Gain  Gain=2
  Product1 : Product  RndMeth=Zero
  Product2 : Product  RndMeth=Zero
  Sum : Sum  Inputs=|++
  A31 : Outport  VectorParamsAs1DForOutWhenUnconnected=off
  wires:
  Product1/1 -> Sum/1
  Demux/4 -> Product2/2
  Sum/1 -> Gain/1
  Demux/3 -> Product1/2
  Demux/1 -> Product1/1
  Gain/1 -> A31/1
  Demux/2 -> Product2/1
  Product2/1 -> Sum/2
  qNormalized/1 -> Demux/1

== system ARIES/C_SB/A32 ==
  qNormalized : Inport
  Demux : Demux
  Gain : Gain  Gain=2
  Product1 : Product  RndMeth=Zero
  Product2 : Product  RndMeth=Zero
  Sum : Sum  Inputs=|-+
  A32 : Outport  VectorParamsAs1DForOutWhenUnconnected=off
  wires:
  Demux/1 -> Product1/1
  Product1/1 -> Sum/1
  Demux/3 -> Product2/1
  Product2/1 -> Sum/2
  Gain/1 -> A32/1
  Demux/4 -> Product2/2
  Sum/1 -> Gain/1
  Demux/2 -> Product1/2
  qNormalized/1 -> Demux/1

== system ARIES/C_SB/A33 ==
  qNormalized : Inport
  Demux : Demux
  Product{,1..3} (4 alike) : Product  RndMeth=Zero
  Sum : Sum  Inputs=+--+
  A33 : Outport  VectorParamsAs1DForOutWhenUnconnected=off
  wires:
  Demux/3 -> Product1/1, Product1/2
  Demux/4 -> Product/1, Product/2
  Sum/1 -> A33/1
  Product/1 -> Sum/4
  Product1/1 -> Sum/3
  Demux/1 -> Product3/1, Product3/2
  qNormalized/1 -> Demux/1
  Product3/1 -> Sum/1
  Demux/2 -> Product2/1, Product2/2
  Product2/1 -> Sum/2

== system ARIES/Control Unit/No Control ==
  SCState : Inport
  Constant : Constant  Value=zeros(3,1)
  Terminator : Terminator
  controlAcc : Outport
  wires:
  SCState/1 -> Terminator/1
  Constant/1 -> controlAcc/1

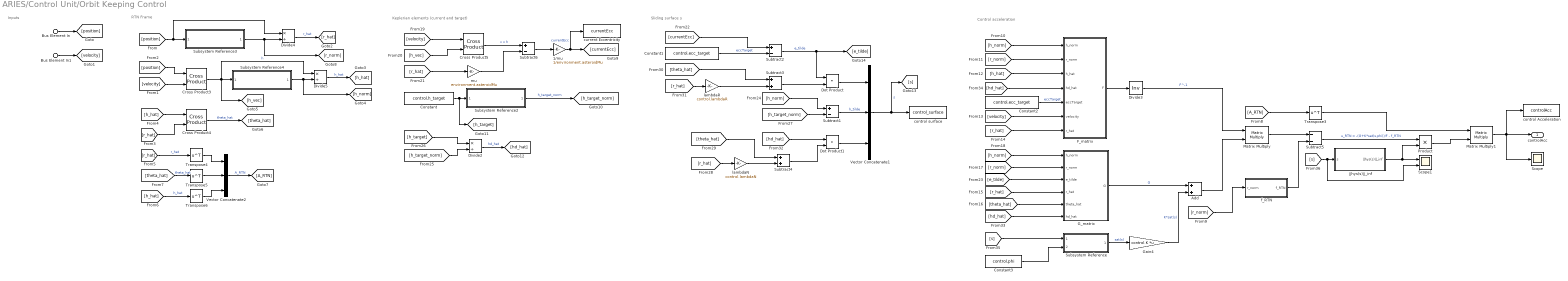
== system ARIES/Control Unit/Orbit Keeping Control ==
  note: Control acceleration
  note: Sliding surface s
  note: Keplerian elements (current and target)
  note: Inputs
  note: RTN Frame
  Bus Element In : Inport  PortName=SCState  Element=position
  Bus Element In1 : Inport  PortName=SCState  Element=velocity
  1/mu : Gain  Gain=1/environment.asteroidMu
  Add : Sum
  Constant : Constant  Value=control.h_target
  Constant1 : Constant  Value=control.ecc_target
  Constant2 : Constant  Value=control.ecc_target
  Constant3 : Constant  Value=control.phi
  Cross Product3 : matrix_library/Cross Product
  Cross Product4 : matrix_library/Cross Product
  Cross Product5 : matrix_library/Cross Product
  Divide2 : Product  Inputs=*/
  Divide3 : Product  Inputs=/  Multiplication=Matrix(*)
  Divide4 : Product  Inputs=*/
  Divide5 : Product  Inputs=*/
  Dot Product : DotProduct  OutDataTypeStr=Inherit: Inherit via internal rule
  Dot Product1 : DotProduct  OutDataTypeStr=Inherit: Inherit via internal rule
  F_matrix : Subsystem
  G_matrix : Subsystem
  Gain4 : Gain  Gain=control.K  Multiplication=Matrix(K*u) (u vector)
  Matrix Multiply : Product  Multiplication=Matrix(*)
  Matrix Multiply1 : Product  Multiplication=Matrix(*)
  Product : Product
  Scope : Scope
  Scope1 : Scope  NumInputPorts=2
  Subsystem Reference : Subsystem  ReferencedSubsystem=saturation
  Subsystem Reference2 : Subsystem  ReferencedSubsystem=VectorNorm
  Subsystem Reference3 : Subsystem  ReferencedSubsystem=VectorNorm
  Subsystem Reference4 : Subsystem  ReferencedSubsystem=VectorNorm
  Subtract1 : Sum  Inputs=+-
  Subtract2 : Sum  Inputs=+-
  Subtract3 : Sum
  Subtract4 : Sum
  Subtract5 : Sum  Inputs=--
  Subtract6 : Sum  Inputs=+-
  Transpose{3..6} (4 alike) : Math  Operator=transpose
  Vector Concatenate1 : Concatenate  NumInputs=3
  Vector Concatenate2 : Concatenate  NumInputs=3  Mode=Multidimensional array
  control Acceleration : ToWorkspace  VariableName=controlAcc  SaveFormat=Timeseries  SampleTime=-1
  control surface : ToWorkspace  VariableName=control_surface  SaveFormat=Timeseries  SampleTime=-1
  current Eccentricity : ToWorkspace  VariableName=currentEcc  SaveFormat=Timeseries  SampleTime=-1
  f_RTN : Subsystem
  lambdaN : Gain  Gain=control.lambdaN
  lambdaR : Gain  Gain=control.lambdaR
  mu : Gain  Gain=environment.asteroidMu
  ||hys(s)||_inf : Subsystem
  controlAcc : Outport
  wires:
  Bus Element In/1 -> [position]
  Bus Element In1/1 -> [velocity]
  Constant/1 -> Subsystem Reference2/1, [h_target]
  Subsystem Reference2/1 -> [h_target_norm]  "h_target_norm"
  Subtract1/1 -> Vector Concatenate1/2  "h_tilde"
  Constant1/1 -> Subtract2/2  "eccTarget"
  Subtract2/1 -> [e_tilde], Dot Product/1  "e_tilde"
  lambdaR/1 -> Subtract3/2
  Subtract3/1 -> Dot Product/2
  Dot Product/1 -> Vector Concatenate1/1
  lambdaN/1 -> Subtract4/2
  Subtract4/1 -> Dot Product1/2
  Dot Product1/1 -> Vector Concatenate1/3
  Vector Concatenate1/1 -> control surface/1, [s]  "s"
  Constant2/1 -> F_matrix/5(eccTarget)  "eccTarget"
  F_matrix/1(F) -> Divide3/1
  Subsystem Reference/1 -> Gain4/1  "sat(s)"
  Gain4/1 -> Add/2  "K*sat(s)"
  Divide3/1 -> Matrix Multiply/1  "F^-1"
  G_matrix/1(G) -> Add/1  "G"
  Add/1 -> Matrix Multiply/2
  Constant3/1 -> Subsystem Reference/2
  Matrix Multiply/1 -> Subtract5/1
  f_RTN/1(f_RTN) -> Subtract5/2
  Subtract5/1 -> Product/1  "u_RTN = -(G+K*sat(s,phi))/F - f_RTN"
  Matrix Multiply1/1 -> control Acceleration/1, controlAcc/1, Scope/1
  Transpose3/1 -> Matrix Multiply1/1
  Subsystem Reference3/1 -> [r_norm], Divide4/2
  [position] -> Divide4/1, Subsystem Reference3/1
  Divide4/1 -> [r_hat]  "r_hat"
  [velocity] -> Cross Product3/2
  [position] -> Cross Product3/1
  Cross Product3/1 -> [h_vec], Divide5/1, Subsystem Reference4/1  "h"
  Subsystem Reference4/1 -> [h_norm], Divide5/2
  Divide5/1 -> [h_hat]  "h_hat"
  [h_hat] -> Cross Product4/1
  [r_hat] -> Cross Product4/2
  Cross Product4/1 -> [theta_hat]  "theta_hat"
  [r_hat] -> Transpose4/1  "r_hat"
  Transpose6/1 -> Vector Concatenate2/3
  [theta_hat] -> Transpose5/1  "theta_hat"
  [h_hat] -> Transpose6/1  "h_hat"
  Transpose5/1 -> Vector Concatenate2/2
  Transpose4/1 -> Vector Concatenate2/1
  Vector Concatenate2/1 -> [A_RTN]  "A_RTN"
  [A_RTN] -> Transpose3/1
  [r_norm] -> f_RTN/1(r_norm)
  [h_norm] -> F_matrix/1(h_norm)
  [r_norm] -> F_matrix/2(r_norm)
  [h_hat] -> F_matrix/3(h_hat)
  [velocity] -> F_matrix/6(velocity)
  [r_hat] -> F_matrix/7(r_hat)
  [r_hat] -> G_matrix/4(r_hat)
  [theta_hat] -> G_matrix/5(theta_hat)
  [r_norm] -> G_matrix/2(r_norm)
  [h_norm] -> G_matrix/1(h_norm)
  [velocity] -> Cross Product5/1
  [h_vec] -> Cross Product5/2
  Cross Product5/1 -> Subtract6/1  "v x h"
  mu/1 -> Subtract6/2
  [r_hat] -> mu/1
  Subtract6/1 -> 1/mu/1
  1/mu/1 -> current Eccentricity/1, [currentEcc]  "currentEcc"
  [currentEcc] -> Subtract2/1
  [e_tilde] -> G_matrix/3(e_tilde)
  [h_norm] -> Subtract1/1
  [h_target_norm] -> Divide2/2
  [h_target] -> Divide2/1
  [h_target_norm] -> Subtract1/2
  [r_hat] -> lambdaN/1
  [theta_hat] -> Subtract4/1
  [theta_hat] -> Subtract3/1
  [r_hat] -> lambdaR/1
  Divide2/1 -> [hd_hat]  "hd_hat"
  [hd_hat] -> Dot Product1/1
  [hd_hat] -> G_matrix/6(hd_hat)
  [hd_hat] -> F_matrix/4(hd_hat)
  [s] -> Subsystem Reference/1
  [s] -> Scope1/2, ||hys(s)||_inf/1(s)
  ||hys(s)||_inf/1(||hys(s)||_inf) -> Scope1/1, Product/2
  Product/1 -> Matrix Multiply1/2

== system ARIES/Control Unit/Waypoint guidance ==
  Bus Element In : Inport  PortName=SCState  Element=position
  Bus Element In1 : Inport  PortName=SCState  Element=velocity
  Constant : Constant  Value=5
  Constant1 : Constant  Value=str2num(simulation.simulationTimeStep)
  Terminator : Terminator
  To Workspace : ToWorkspace  VariableName=currentWaypointIdx  SaveFormat=Timeseries  SampleTime=-1
  To Workspace1 : ToWorkspace  Commented=on  VariableName=dvArrLog  SaveFormat=Timeseries  SampleTime=-1
  To Workspace2 : ToWorkspace  Commented=on  VariableName=dvDepLog  SaveFormat=Timeseries  SampleTime=-1
  To Workspace3 : ToWorkspace  VariableName=rrLog  SaveFormat=Timeseries  SampleTime=-1
  To Workspace4 : ToWorkspace  Commented=on  VariableName=dvCmdLog  SaveFormat=Timeseries  SampleTime=-1
  To Workspace5 : ToWorkspace  VariableName=dtUpdLog  SaveFormat=Timeseries  SampleTime=-1
  To Workspace6 : ToWorkspace  Commented=on  VariableName=rr2Log  SaveFormat=Timeseries  SampleTime=-1
  Waypoint State Machine : Stateflow chart  TreatAsAtomicUnit=on  SystemSampleTime=0.1
      settings: PortSchema="{\"entries\":[{\"content\":{\"sides\":[{\"content\":{\"connectorIds\":[\"In1\",\"In2\",\"In3\",\"In4\"]},\"type\":\"ConnectorPlacement.EquallySpacedRectSide\",\"uuid\":\"8823d6aa-5e29-4f04-bb66-b46bb85996cd\"},{\"content\":{\"connectorIds\":[\"Out2\",\"Out1\",\"Out3\",\"Out4\",\"Out5\",\"Out6\",\"Out7\",\"Out8\",\"Out9\"],\"side\":\"RIGHT\"},\"type\":\"ConnectorPlacement.EquallySpacedRectSide\",\"uuid\":\"c48127e7-4501-4f1c-8b72-742d4140b278\"},{\"content\":{\"side\":\"TOP\"},\"type\":\"ConnectorPlacement.EquallySpacedRectSide\",\"uuid\":\"d020961e-874c-481b-8f7d-7308bf4e188b\"}]},\"type\":\"ConnectorPlacement.EquallySpacedConnector\",\"uuid\":\"10347344-04aa-4deb-92ed-16b0d69d7c68\"}],\"packageUris\":[\"http://schema.mathworks.com/mf0/Connector/R2020b\"],\"version\":\"1.0\"}"
  control Acceleration : ToWorkspace  VariableName=controlAcc  SaveFormat=Timeseries  SampleTime=-1
  controlAcc : Outport
  wires:
  Waypoint State Machine/2(controlAcc) -> control Acceleration/1, controlAcc/1
  Waypoint State Machine/1(currentWpIdx) -> To Workspace/1
  Waypoint State Machine/3(burnActive) -> Terminator/1
  Bus Element In/1 -> Waypoint State Machine/3(SCPosition)
  Bus Element In1/1 -> Waypoint State Machine/4(SCVelocity)
  Constant1/1 -> Waypoint State Machine/1(dtSim)
  Constant/1 -> Waypoint State Machine/2(tBurn)
  Waypoint State Machine/4(dvArrLog) -> To Workspace1/1
  Waypoint State Machine/5(dvDepLog) -> To Workspace2/1
  Waypoint State Machine/6(rTraj) -> To Workspace3/1
  Waypoint State Machine/7(dvCmd) -> To Workspace4/1
  Waypoint State Machine/8(rTraj2) -> To Workspace6/1
  Waypoint State Machine/9(dt_new) -> To Workspace5/1

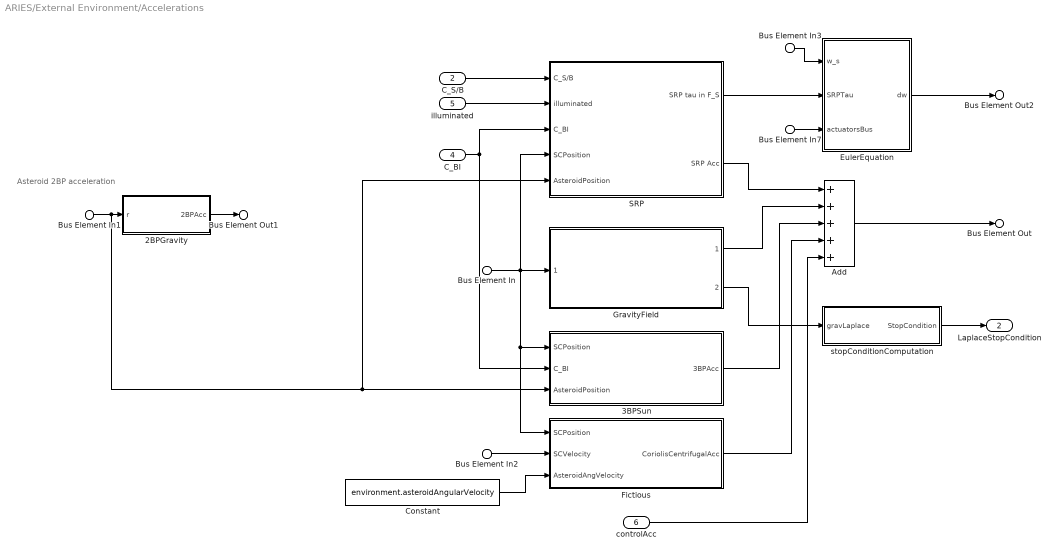
== system ARIES/External Environment/Accelerations ==
  note: Asteroid 2BP acceleration
  Bus Element In1 : Inport  PortName=AsteroidState  Element=position
  C_S/B : Inport  Port=2
  Bus Element In : Inport  Port=3  PortName=SCState  Element=position
  Bus Element In2 : Inport  Port=3  PortName=SCState  Element=velocity
  Bus Element In3 : Inport  Port=3  PortName=SCState  Element=ang_velocity
  C_BI : Inport  Port=4
  illuminated : Inport  Port=5
  controlAcc : Inport  Port=6
  Bus Element In7 : Inport  Port=7  PortName=actuatorsBus
  2BPGravity : Subsystem
  3BPSun : Subsystem
  Add : Sum  Inputs=5
  Constant : Constant  Value=environment.asteroidAngularVelocity
  EulerEquation : Subsystem
  Fictious : Subsystem
  GravityField : Subsystem  ReferencedSubsystem=GravityField
  SRP : Subsystem
  stopConditionComputation : Subsystem
  Bus Element Out : Outport  PortName=Accelerations  Element=SC_lin
  Bus Element Out1 : Outport  PortName=Accelerations  Element=asteroid_lin
  Bus Element Out2 : Outport  PortName=Accelerations  Element=SC_ang
  LaplaceStopCondition : Outport  Port=2
  wires:
  Bus Element In1/1 -> 3BPSun/3(AsteroidPosition), SRP/5(AsteroidPosition), 2BPGravity/1(r)
  C_BI/1 -> SRP/3(C_BI), 3BPSun/2(C_BI)
  Bus Element In/1 -> Fictious/1(SCPosition), 3BPSun/1(SCPosition), SRP/4(SCPosition), GravityField/1
  illuminated/1 -> SRP/2(illuminated)
  C_S/B/1 -> SRP/1(C_S/B)
  2BPGravity/1(2BPAcc) -> Bus Element Out1/1
  GravityField/2 -> stopConditionComputation/1(gravLaplace)
  Add/1 -> Bus Element Out/1
  GravityField/1 -> Add/2
  stopConditionComputation/1(StopCondition) -> LaplaceStopCondition/1
  EulerEquation/1(dw) -> Bus Element Out2/1
  Bus Element In2/1 -> Fictious/2(SCVelocity)
  Constant/1 -> Fictious/3(AsteroidAngVelocity)
  Fictious/1(CoriolisCentrifugalAcc) -> Add/4
  controlAcc/1 -> Add/5
  Bus Element In3/1 -> EulerEquation/1(w_s)
  SRP/1(SRP tau in F_S) -> EulerEquation/2(SRPTau)
  Bus Element In7/1 -> EulerEquation/3(actuatorsBus)
  SRP/2(SRP Acc) -> Add/1
  3BPSun/1(3BPAcc) -> Add/3

== system ARIES/External Environment/DerivativeStateAssembly ==
  Bus Element In : Inport  PortName=SCState  Element=velocity
  Bus Element In5 : Inport  PortName=SCState  Element=q_SB
  Bus Element In6 : Inport  PortName=SCState  Element=ang_velocity
  C_S/B : Inport  Port=2
  Bus Element In1 : Inport  Port=3  PortName=AsteroidState  Element=velocity
  Bus Element In3 : Inport  Port=4  PortName=Accelerations  Element=SC_lin
  Bus Element In4 : Inport  Port=4  PortName=Accelerations  Element=SC_ang
  Bus Element In2 : Inport  Port=4  PortName=Accelerations  Element=asteroid_lin
  Vector Concatenate : Concatenate  NumInputs=6
  dq/dt : Subsystem
  dY : Outport
  wires:
  Vector Concatenate/1 -> dY/1
  Bus Element In/1 -> Vector Concatenate/1
  Bus Element In1/1 -> Vector Concatenate/5
  Bus Element In3/1 -> Vector Concatenate/2
  Bus Element In2/1 -> Vector Concatenate/6
  dq/dt/1(dQ) -> Vector Concatenate/3
  Bus Element In4/1 -> Vector Concatenate/4
  Bus Element In5/1 -> dq/dt/1(q_SB)
  Bus Element In6/1 -> dq/dt/3(SCAngVel)
  C_S/B/1 -> dq/dt/2(C_S/B)

== system ARIES/External Environment/InitialConditionAssembly ==
  AsteroidState_position0 : Constant  Value=init.asteroidPosition
  AsteroidState_velocity0 : Constant  Value=init.asteroidVelocity
  SCState_ang_velocity0 : Constant  Value=init.scAngularVel
  SCState_position0 : Constant  Value=init.scPosition
  SCState_qSB0 : Constant  Value=init.quaternion
  SCState_velocity0 : Constant  Value=init.scVelocity
  Vector Concatenate : Concatenate  NumInputs=6
  Y0 : Outport
  wires:
  Vector Concatenate/1 -> Y0/1
  SCState_position0/1 -> Vector Concatenate/1
  SCState_velocity0/1 -> Vector Concatenate/2
  SCState_qSB0/1 -> Vector Concatenate/3
  SCState_ang_velocity0/1 -> Vector Concatenate/4
  AsteroidState_position0/1 -> Vector Concatenate/5
  AsteroidState_velocity0/1 -> Vector Concatenate/6

== system ARIES/External Environment/OrbitCounter ==
  Y0 : Inport
  Bus Element In2 : Inport  Port=2  PortName=SCState  Element=position
  Compare To Constant : simulink/Logic and Bit Operations/Compare To Constant  relop=<=  const=simulation.startPosThreshold  OutDataTypeStr=boolean
  Compare To Constant1 : simulink/Logic and Bit Operations/Compare To Constant  relop=>=  const=simulation.nOrbits  OutDataTypeStr=boolean
  Memory : Memory
  Selector : Selector  InputPortWidth=19  IndexOptions=Index vector (dialog)  Indices=1:3  OutputSizes=1
  Stop Simulation : Stop
  Subsystem Reference : Subsystem  ReferencedSubsystem=VectorNorm
  Subtract : Sum  Inputs=+-
  To Workspace : ToWorkspace  VariableName=nOrbits  SaveFormat=Timeseries  SampleTime=-1
  Triggered Subsystem : Subsystem  TreatAsAtomicUnit=on
  wires:
  Y0/1 -> Selector/1
  Bus Element In2/1 -> Subtract/2
  Subtract/1 -> Subsystem Reference/1
  Subsystem Reference/1 -> Compare To Constant/1
  Compare To Constant/1 -> Triggered Subsystem/Trigger
  Triggered Subsystem/1(Out1) -> Memory/1
  Memory/1 -> To Workspace/1, Compare To Constant1/1, Triggered Subsystem/1(In1)
  Selector/1 -> Subtract/1
  Compare To Constant1/1 -> Stop Simulation/1

== system ARIES/External Environment/StateToBusConversion ==
  Y : Inport
  Quaternion Normalize : sharedutil/Quaternion Normalize  aMode=aMode
  Selector1 : Selector  InputPortWidth=19  IndexOptions=Index vector (dialog)  Indices=[4:6]  OutputSizes=1
  Selector2 : Selector  InputPortWidth=19  IndexOptions=Index vector (dialog)  Indices=[7:10]  OutputSizes=1
  Selector3 : Selector  InputPortWidth=19  IndexOptions=Index vector (dialog)  Indices=[11:13]  OutputSizes=1
  Selector4 : Selector  InputPortWidth=19  IndexOptions=Index vector (dialog)  Indices=[14:16]  OutputSizes=1
  Selector5 : Selector  InputPortWidth=19  IndexOptions=Index vector (dialog)  Indices=[1:3]  OutputSizes=1
  Selector6 : Selector  InputPortWidth=19  IndexOptions=Index vector (dialog)  Indices=[17:19]  OutputSizes=1
  Bus Element Out4 : Outport  PortName=AsteroidState  Element=position
  Bus Element Out5 : Outport  PortName=AsteroidState  Element=velocity
  Bus Element Out : Outport  Port=2  PortName=SCState  Element=position
  Bus Element Out1 : Outport  Port=2  PortName=SCState  Element=velocity
  Bus Element Out2 : Outport  Port=2  PortName=SCState  Element=q_SB
  Bus Element Out3 : Outport  Port=2  PortName=SCState  Element=ang_velocity
  wires:
  Y/1 -> Selector1/1, Selector5/1, Selector2/1, Selector6/1, Selector4/1, Selector3/1
  Selector5/1 -> Bus Element Out/1
  Selector1/1 -> Bus Element Out1/1
  Selector2/1 -> Quaternion Normalize/1
  Selector3/1 -> Bus Element Out3/1
  Selector4/1 -> Bus Element Out4/1
  Selector6/1 -> Bus Element Out5/1
  Quaternion Normalize/1 -> Bus Element Out2/1

== system ARIES/Actuators/Reaction wheels + thrusters/hr_sat ==
  hr : Inport
  Constant : Constant  Value=actuators.rw.hrMax_total
  Product : Product  Inputs=**/
  Subsystem Reference : Subsystem  ReferencedSubsystem=VectorNorm
  Switch : Switch  Criteria=u2 > Threshold  Threshold=actuators.rw.hrMax_total  SaturateOnIntegerOverflow=off  InputSameDT=off
  hr_sat : Outport
  wires:
  hr/1 -> Product/2, Switch/3, Subsystem Reference/1
  Subsystem Reference/1 -> Switch/2, Product/3
  Switch/1 -> hr_sat/1
  Product/1 -> Switch/1
  Constant/1 -> Product/1

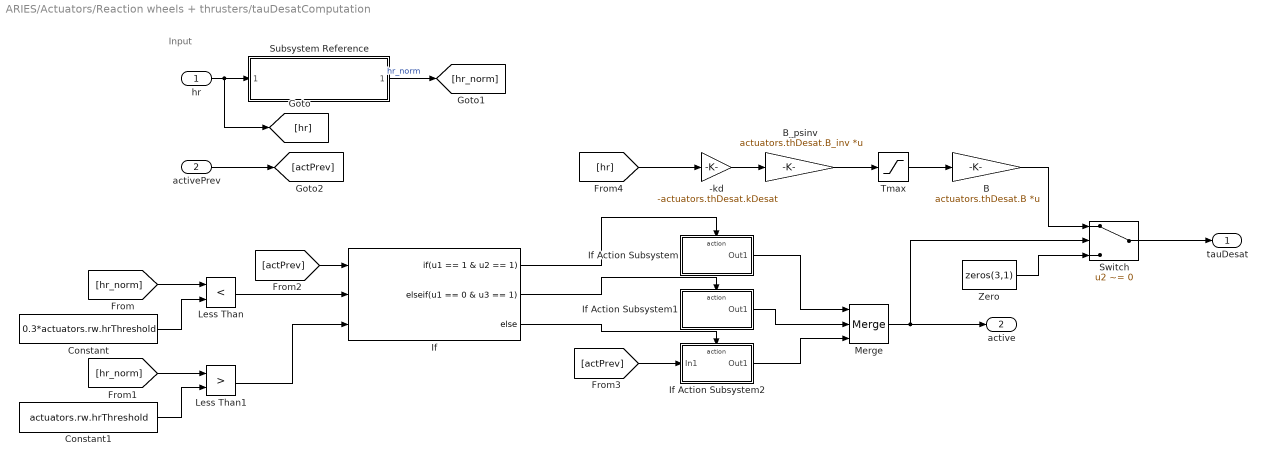
== system ARIES/Actuators/Reaction wheels + thrusters/tauDesatComputation ==
  note: Input
  hr : Inport
  activePrev : Inport  Port=2
  -kd : Gain  Gain=-actuators.thDesat.kDesat
  B : Gain  Gain=actuators.thDesat.B  Multiplication=Matrix(K*u) (u vector)
  B_psinv : Gain  Gain=actuators.thDesat.B_inv  Multiplication=Matrix(K*u) (u vector)
  Constant : Constant  Value=0.3*actuators.rw.hrThreshold
  Constant1 : Constant  Value=actuators.rw.hrThreshold
  If : If  NumInputs=3  IfExpression=u1 == 1 & u2 == 1  ElseIfExpressions=u1 == 0 & u3 == 1
  If Action Subsystem : Subsystem  TreatAsAtomicUnit=on
  If Action Subsystem1 : Subsystem  TreatAsAtomicUnit=on
  If Action Subsystem2 : Subsystem  TreatAsAtomicUnit=on
  Less Than : RelationalOperator  Operator=<  OutDataTypeStr=boolean  RndMeth=Simplest  InputSameDT=off
  Less Than1 : RelationalOperator  Operator=>  OutDataTypeStr=boolean  RndMeth=Simplest  InputSameDT=off
  Merge : Merge  Inputs=3  InitialOutput=0
  Subsystem Reference : Subsystem  ReferencedSubsystem=VectorNorm
  Switch : Switch  Criteria=u2 ~= 0  SaturateOnIntegerOverflow=off  InputSameDT=off
  Tmax : Saturate  UpperLimit=actuators.thDesat.Tmax*ones(8,1)  LowerLimit=zeros(8,1)
  Zero : Constant  Value=zeros(3,1)  OutDataTypeStr=Inherit: Inherit via back propagation
  tauDesat : Outport
  active : Outport  Port=2
  wires:
  hr/1 -> [hr], Subsystem Reference/1
  Subsystem Reference/1 -> [hr_norm]  "hr_norm"
  [hr_norm] -> Less Than/1
  Constant/1 -> Less Than/2
  Less Than/1 -> If/2
  Constant1/1 -> Less Than1/2
  [hr_norm] -> Less Than1/1
  Less Than1/1 -> If/3
  activePrev/1 -> [actPrev]
  [actPrev] -> If/1
  Merge/1 -> active/1, Switch/2
  If/1 -> If Action Subsystem/Action
  If Action Subsystem/1(Out1) -> Merge/1
  If Action Subsystem1/1(Out1) -> Merge/2
  If/2 -> If Action Subsystem1/Action
  If Action Subsystem2/1(Out1) -> Merge/3
  If/3 -> If Action Subsystem2/Action
  [actPrev] -> If Action Subsystem2/1(In1)
  Switch/1 -> tauDesat/1
  Zero/1 -> Switch/3
  B/1 -> Switch/1
  Tmax/1 -> B/1
  B_psinv/1 -> Tmax/1
  -kd/1 -> B_psinv/1
  [hr] -> -kd/1

== system ARIES/Attitude Control/Attitude error quat copy/If Action Subsystem ==
  In1 : Inport
  Action Port : ActionPort
  Gain : Gain  Gain=-1
  Out1 : Outport
  wires:
  In1/1 -> Gain/1
  Gain/1 -> Out1/1

== system ARIES/Attitude Control/Attitude error quat copy/If Action Subsystem1 ==
  In1 : Inport
  sign_state : Inport  Port=2
  Action Port : ActionPort
  Product : Product
  Out1 : Outport
  wires:
  In1/1 -> Product/1
  Product/1 -> Out1/1
  sign_state/1 -> Product/2

== system ARIES/Attitude Control/Attitude error quat copy/If Action Subsystem2 ==
  In1 : Inport
  Action Port : ActionPort
  Out1 : Outport
  wires:
  In1/1 -> Out1/1

== system ARIES/Attitude Control/Variant Subsystem/INERTIAL ==
  C_SB : Inport
  Constant1 : Constant  Value=environment.asteroidAngularVelocity
  Constant3 : Constant  Value=eye(3)
  Direction Cosine Matrix to Quaternions : sharedtransform/Direction Cosine Matrix  to Quaternions  aMode=0  action=None  tolerance=eps(2)
      settings: LibrarySourceBlock=|
      | aerolibtransform2/Direction Cosine Matrix
      | to Quaternions
  Matrix Multiply3 : Product  Multiplication=Matrix(*)
  q_target : Outport
  A_target : Outport  Port=2
  w_target : Outport  Port=3
  wires:
  Constant3/1 -> Direction Cosine Matrix to Quaternions/1, A_target/1  "A_target"
  Direction Cosine Matrix to Quaternions/1 -> q_target/1
  Constant1/1 -> Matrix Multiply3/2
  Matrix Multiply3/1 -> w_target/1
  C_SB/1 -> Matrix Multiply3/1

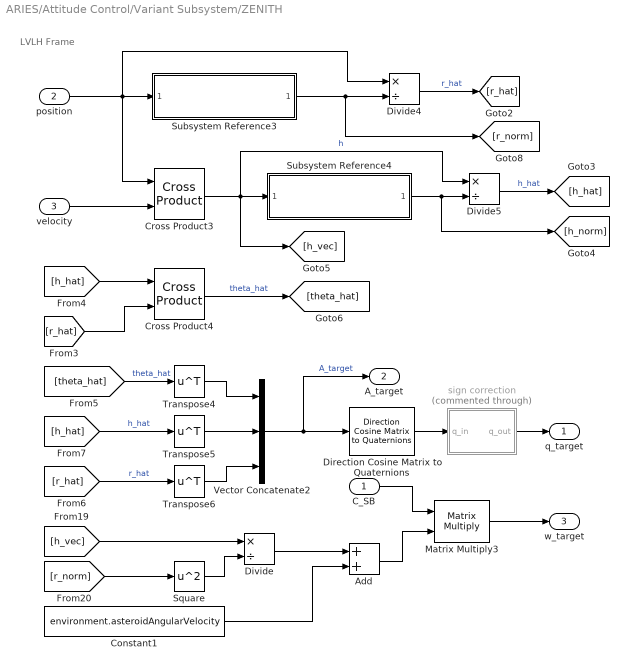
== system ARIES/Attitude Control/Variant Subsystem/ZENITH ==
  note: LVLH Frame
  C_SB : Inport
  position : Inport  Port=2
  velocity : Inport  Port=3
  Add : Sum
  Constant1 : Constant  Value=environment.asteroidAngularVelocity
  Cross Product3 : matrix_library/Cross Product
  Cross Product4 : matrix_library/Cross Product
  Direction Cosine Matrix to Quaternions : sharedtransform/Direction Cosine Matrix  to Quaternions  aMode=0  action=None  tolerance=eps(2)
      settings: LibrarySourceBlock=|
      | aerolibtransform2/Direction Cosine Matrix
      | to Quaternions
  Divide : Product  Inputs=*/
  Divide4 : Product  Inputs=*/
  Divide5 : Product  Inputs=*/
  Matrix Multiply3 : Product  Multiplication=Matrix(*)
  Square : Math  Operator=square
  Subsystem Reference3 : Subsystem  ReferencedSubsystem=VectorNorm
  Subsystem Reference4 : Subsystem  ReferencedSubsystem=VectorNorm
  Transpose4 : Math  Operator=transpose
  Transpose5 : Math  Operator=transpose
  Transpose6 : Math  Operator=transpose
  Vector Concatenate2 : Concatenate  NumInputs=3  Mode=Multidimensional array  ConcatenateDimension=2
  sign correction : Subsystem  Commented=through
  q_target : Outport
  A_target : Outport  Port=2
  w_target : Outport  Port=3
  wires:
  Divide5/1 -> [h_hat]  "h_hat"
  Transpose5/1 -> Vector Concatenate2/2
  Square/1 -> Divide/2
  position/1 -> Cross Product3/1, Divide4/1, Subsystem Reference3/1
  Subsystem Reference3/1 -> [r_norm], Divide4/2
  [h_vec] -> Divide/1
  Subsystem Reference4/1 -> [h_norm], Divide5/2
  Direction Cosine Matrix to Quaternions/1 -> sign correction/1(q_in)
  [theta_hat] -> Transpose4/1  "theta_hat"
  [h_hat] -> Transpose5/1  "h_hat"
  [r_norm] -> Square/1
  Vector Concatenate2/1 -> Direction Cosine Matrix to Quaternions/1, A_target/1  "A_target"
  Constant1/1 -> Add/2
  Cross Product4/1 -> [theta_hat]  "theta_hat"
  Transpose6/1 -> Vector Concatenate2/3
  Divide4/1 -> [r_hat]  "r_hat"
  Transpose4/1 -> Vector Concatenate2/1
  Matrix Multiply3/1 -> w_target/1
  [r_hat] -> Cross Product4/2
  Cross Product3/1 -> [h_vec], Divide5/1, Subsystem Reference4/1  "h"
  Add/1 -> Matrix Multiply3/2
  velocity/1 -> Cross Product3/2
  [h_hat] -> Cross Product4/1
  C_SB/1 -> Matrix Multiply3/1
  [r_hat] -> Transpose6/1  "r_hat"
  Divide/1 -> Add/1
  sign correction/1(q_out) -> q_target/1
